simulink library "multicopterNDI_lib"  (R2018b)
settings: Solver=VariableStepAuto  StartTime=0.0  StopTime=10.0  RelTol=1e-3
undefined symbols (not defined in the file or in its folder): cntrl, DiscIntNeverNeededParam
libraries: ndi_lib x5, axes_transformation_lib x1
settings Model: Creator=Ybeyer  LastModifiedBy=yannic
settings SFSimCC: SimUseLocalCustomCode=off
settings RTWCC: RTWUseLocalCustomCode=off
settings CodeAppCC: StateflowObjectComments=on

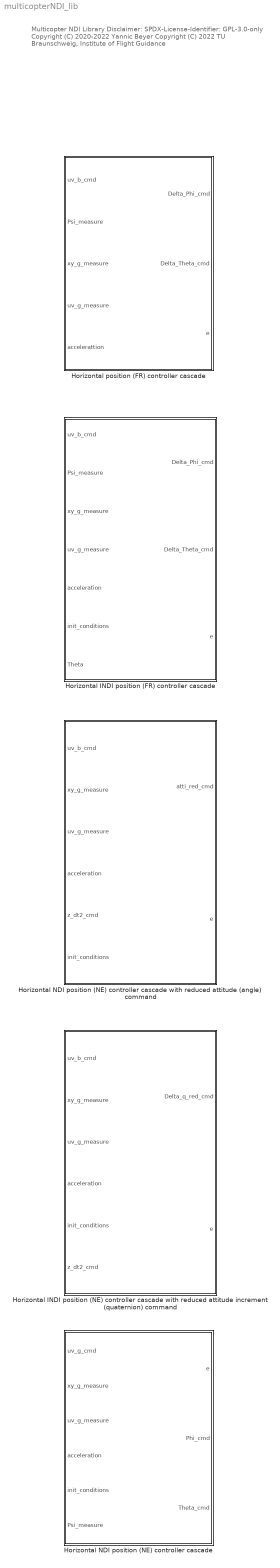
== system multicopterNDI_lib ==
  note: Multicopter NDI Library
      |
      | Disclaimer:
      | SPDX-License-Identifier: GPL-3.0-only
      |
      | Copyright (C) 2020-2022 Yannic Beyer
      | Copyright (C) 2022 TU Braunschweig, Institute of Flight Guidance
  Horizontal INDI position (FR) controller cascade : Subsystem  mask{time_constant_V=cntrl.rm.u.T, V_dt_max=inf, K_xyuv=cntrl.Kpos, K_int_xy=zeros(2,2), Phi_cmd_max=pi/4, Theta_cmd_max=pi/4}
      mask prompts: time_constant_V "commanded velocity time constant, in s"; V_dt_max "maximum commanded acceleration"; K_xyuv "controller matrix [e_x,e_y,e_u,e_v] -> [x_ddt,y_ddt]_cmd"; K_int_xy "I controller matrix [int_e_x,int_e_y] -> [x_ddt,y_ddt]_cmd"; Phi_cmd_max "Maximum commanded roll angle"; Theta_cmd_max "Maximum commanded picth angle"
      mask DialogControl DescGroupVar Prompt: Horizontal position controller cascade
      mask DialogControl DescTextVar Prompt: The commanded velocity is filtered and the control error is converted into desired accerlations in x_b and y_b direction. The commanded accelerations are converted into commanded roll and pitch angles.
  Horizontal INDI position (NE) controller cascade with reduced attitude increment (quaternion) command : Subsystem  mask{time_constant_V=cntrl.rm.u.T, V_dt_max=cntrl.rm.uv_dt_max, K_xyuv=cntrl.Kpos, tilt_angle_max=cntrl.rm.Phi_max, e_xy_max=cntrl.e_xy_max}
      mask prompts: time_constant_V "commanded velocity time constant, in s"; V_dt_max "maximum commanded acceleration"; K_xyuv "controller matrix [e_x,e_y,e_u,e_v] -> [x_ddt,y_ddt]_cmd"; tilt_angle_max "Maximum commanded tilt angle"; e_xy_max "Maximum position error (to limit maximum velocity due to controller)"
      mask DialogControl DescGroupVar Prompt: Horizontal position controller cascade
      mask DialogControl DescTextVar Prompt: The commanded velocity is filtered and the control error is converted into desired accerlations in x_b and y_b direction. The commanded accelerations are converted into commanded roll and pitch angles.
  Horizontal NDI position (NE) controller cascade : Subsystem  mask{time_constant_V=cntrl.rm.u.T, V_dt_max=inf, K_xyuv=cntrl.Kpos, K_int_xy=zeros(2,2), Phi_cmd_max=pi/4, Theta_cmd_max=pi/4}
      mask prompts: time_constant_V "commanded velocity time constant, in s"; V_dt_max "maximum commanded acceleration"; K_xyuv "controller matrix [e_x,e_y,e_u,e_v] -> [x_ddt,y_ddt]_cmd"; K_int_xy "I controller matrix [int_e_x,int_e_y] -> [x_ddt,y_ddt]_cmd"; Phi_cmd_max "Maximum commanded roll angle"; Theta_cmd_max "Maximum commanded picth angle"
      mask DialogControl DescGroupVar Prompt: Horizontal position controller cascade (commanding velocities/positions in north/east (NE) direction)
      mask DialogControl DescTextVar Prompt: The commanded velocity is filtered and the control error is converted into desired accerlations in x_b and y_b direction. The commanded accelerations are converted into commanded roll and pitch angles.
  Horizontal NDI position (NE) controller cascade with reduced attitude (angle) command : Subsystem  mask{time_constant_V=cntrl.rm.u.T, V_dt_max=cntrl.rm.uv_dt_max, K_xyuv=cntrl.Kpos, K_int_xy=cntrl.Kpos_I, e_xy_max=cntrl.e_xy_max}
      mask prompts: time_constant_V "commanded velocity time constant, in s"; V_dt_max "maximum commanded acceleration"; K_xyuv "controller matrix [e_x,e_y,e_u,e_v] -> [x_ddt,y_ddt]_cmd"; K_int_xy "I controller matrix [int_e_x,int_e_y] -> [x_ddt,y_ddt]_cmd"; e_xy_max "Maximum controller position error (to limit maximum velocity due to controller)"
      mask DialogControl DescGroupVar Prompt: Horizontal position controller cascade
      mask DialogControl DescTextVar Prompt: The commanded velocity is filtered and the control error is converted into desired accerlations in x_g and y_g direction. The commanded accelerations are converted into commanded to reduced attitude angles.
  Horizontal position (FR) controller cascade : Subsystem  mask{time_constant_V=1, V_dt_max=inf, K_xyuv=zeros(2,4), K_int_xy=zeros(2,2), Phi_cmd_max=pi/4, Theta_cmd_max=pi/4}
      mask prompts: time_constant_V "commanded velocity time constant, in s"; V_dt_max "maximum commanded acceleration"; K_xyuv "controller matrix [e_x,e_y,e_u,e_v] -> [x_ddt,y_ddt]_cmd"; K_int_xy "I controller matrix [int_e_x,int_e_y] -> [x_ddt,y_ddt]_cmd"; Phi_cmd_max "Maximum commanded roll angle"; Theta_cmd_max "Maximum commanded picth angle"
      mask DialogControl DescGroupVar Prompt: Horizontal position controller cascade
      mask DialogControl DescTextVar Prompt: The commanded velocity is filtered and the control error is converted into desired accerlations in x_b and y_b direction. The commanded accelerations are converted into commanded roll and pitch angles.

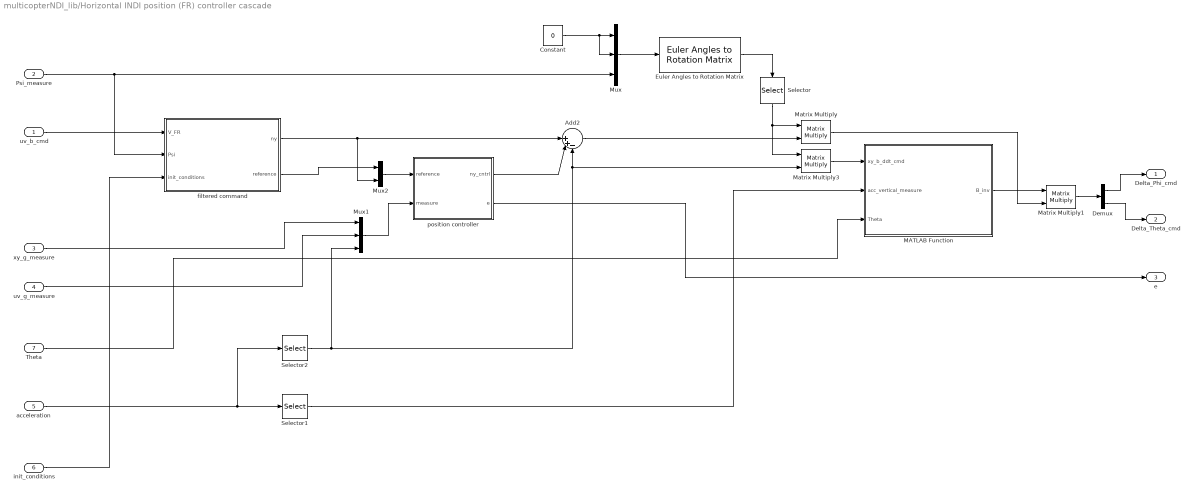
== system multicopterNDI_lib/Horizontal INDI position (FR) controller cascade ==
  uv_b_cmd : Inport
  Psi_measure : Inport  Port=2
  xy_g_measure : Inport  Port=3
  uv_g_measure : Inport  Port=4
  acceleration : Inport  Port=5
  init_conditions : Inport  Port=6
  Theta : Inport  Port=7
  Add2 : Sum  Inputs=||++-
  Constant : Constant  Value=0  OutDataTypeStr=Inherit: Inherit via back propagation
  Demux : Demux  Outputs=2
  Euler Angles to Rotation Matrix : axes_transformation_lib/Euler Angles to Rotation Matrix  SystemSampleTime=-1
      settings: SourceProductName=LADAC
  MATLAB Function : MATLAB Function  TreatAsAtomicUnit=on
  Matrix Multiply : Product  Multiplication=Matrix(*)
  Matrix Multiply1 : Product  Multiplication=Matrix(*)
  Matrix Multiply3 : Product  Multiplication=Matrix(*)
  Mux : Mux  Inputs=3
  Mux1 : Mux  Inputs=3
  Mux2 : Mux  Inputs=2
  Selector : Selector  NumberOfDimensions=2  InputPortWidth=[3,3]  IndexOptions=Index vector (dialog),Index vector (dialog)  Indices=[1:2],[1:2]  OutputSizes=1,1
  Selector1 : Selector  InputPortWidth=3  IndexOptions=Index vector (dialog)  Indices=3  OutputSizes=1
  Selector2 : Selector  InputPortWidth=3  IndexOptions=Index vector (dialog)  Indices=[1,2]  OutputSizes=1
  filtered command : Subsystem
  position controller : Subsystem
  Delta_Phi_cmd : Outport
  Delta_Theta_cmd : Outport  Port=2
  e : Outport  Port=3
  wires:
  init_conditions/1 -> filtered command/3(init_conditions)
  Mux2/1 -> position controller/1(reference)
  position controller/2(e) -> e/1
  Matrix Multiply1/1 -> Demux/1
  Demux/2 -> Delta_Theta_cmd/1
  Demux/1 -> Delta_Phi_cmd/1
  MATLAB Function/1(B_inv) -> Matrix Multiply1/1
  Selector2/1 -> Mux1/3, Add2/3, Matrix Multiply3/2
  Selector1/1 -> MATLAB Function/2(acc_vertical_measure)
  Euler Angles to Rotation Matrix/1 -> Selector/1
  Matrix Multiply/1 -> Matrix Multiply1/2
  Constant/1 -> Mux/1, Mux/2
  Mux/1 -> Euler Angles to Rotation Matrix/1
  Psi_measure/1 -> filtered command/2(Psi), Mux/3
  filtered command/2(reference) -> Mux2/1
  uv_b_cmd/1 -> filtered command/1(V_FR)
  acceleration/1 -> Selector2/1, Selector1/1
  position controller/1(ny_cntrl) -> Add2/2
  filtered command/1(ny) -> Mux2/2, Add2/1
  Add2/1 -> Matrix Multiply/2
  Mux1/1 -> position controller/2(measure)
  xy_g_measure/1 -> Mux1/1
  uv_g_measure/1 -> Mux1/2
  Matrix Multiply3/1 -> MATLAB Function/1(xy_b_ddt_cmd)
  Selector/1 -> Matrix Multiply3/1, Matrix Multiply/1
  Theta/1 -> MATLAB Function/3(Theta)

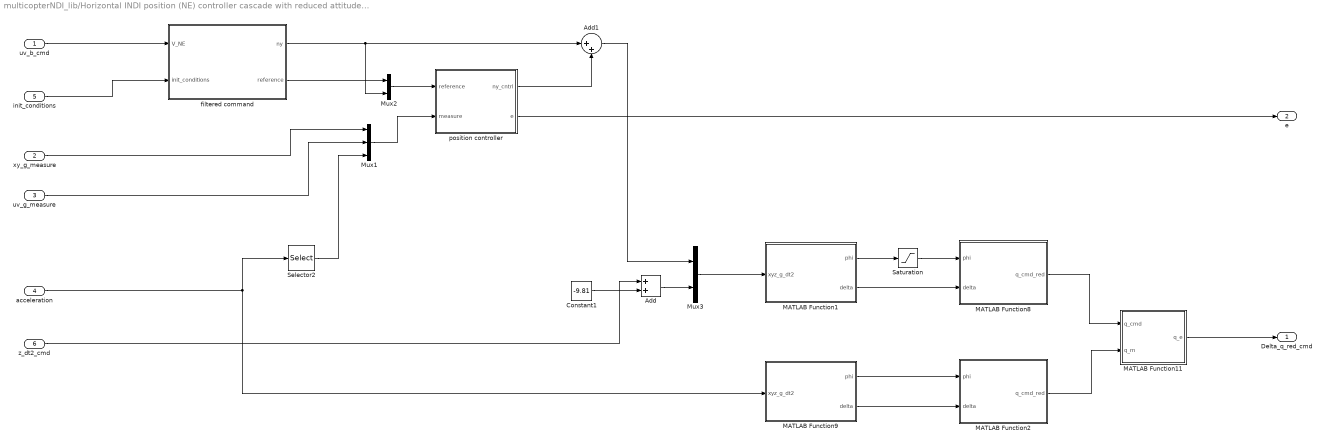
== system multicopterNDI_lib/Horizontal INDI position (NE) controller cascade with reduced attitude increment (quaternion) command ==
  uv_b_cmd : Inport
  xy_g_measure : Inport  Port=2
  uv_g_measure : Inport  Port=3
  acceleration : Inport  Port=4
  init_conditions : Inport  Port=5
  z_dt2_cmd : Inport  Port=6
  Add : Sum
  Add1 : Sum  Inputs=|++
  Constant1 : Constant  Value=-9.81  OutDataTypeStr=single
  MATLAB Function1 : MATLAB Function  TreatAsAtomicUnit=on
  MATLAB Function11 : MATLAB Function  TreatAsAtomicUnit=on
  MATLAB Function2 : MATLAB Function  TreatAsAtomicUnit=on
  MATLAB Function8 : MATLAB Function  TreatAsAtomicUnit=on
  MATLAB Function9 : MATLAB Function  TreatAsAtomicUnit=on
  Mux1 : Mux  Inputs=3
  Mux2 : Mux  Inputs=2
  Mux3 : Mux  Inputs=2
  Saturation : Saturate  UpperLimit=tilt_angle_max  LowerLimit=0
  Selector2 : Selector  InputPortWidth=3  IndexOptions=Index vector (dialog)  Indices=[1,2]  OutputSizes=1
  filtered command : Subsystem
  position controller : Subsystem
  Delta_q_red_cmd : Outport
  e : Outport  Port=2
  wires:
  uv_g_measure/1 -> Mux1/2
  xy_g_measure/1 -> Mux1/1
  Mux1/1 -> position controller/2(measure)
  filtered command/1(ny) -> Add1/1, Mux2/2
  uv_b_cmd/1 -> filtered command/1(V_NE)
  filtered command/2(reference) -> Mux2/1
  Selector2/1 -> Mux1/3
  position controller/2(e) -> e/1
  Mux2/1 -> position controller/1(reference)
  init_conditions/1 -> filtered command/2(init_conditions)
  z_dt2_cmd/1 -> Add/1
  MATLAB Function1/1(phi) -> Saturation/1
  MATLAB Function1/2(delta) -> MATLAB Function8/2(delta)
  position controller/1(ny_cntrl) -> Add1/2
  acceleration/1 -> MATLAB Function9/1(xyz_g_dt2), Selector2/1
  MATLAB Function9/1(phi) -> MATLAB Function2/1(phi)
  MATLAB Function9/2(delta) -> MATLAB Function2/2(delta)
  MATLAB Function8/1(q_cmd_red) -> MATLAB Function11/1(q_cmd)
  MATLAB Function2/1(q_cmd_red) -> MATLAB Function11/2(q_m)
  MATLAB Function11/1(q_e) -> Delta_q_red_cmd/1
  Add/1 -> Mux3/2
  Constant1/1 -> Add/2
  Mux3/1 -> MATLAB Function1/1(xyz_g_dt2)
  Add1/1 -> Mux3/1
  Saturation/1 -> MATLAB Function8/1(phi)

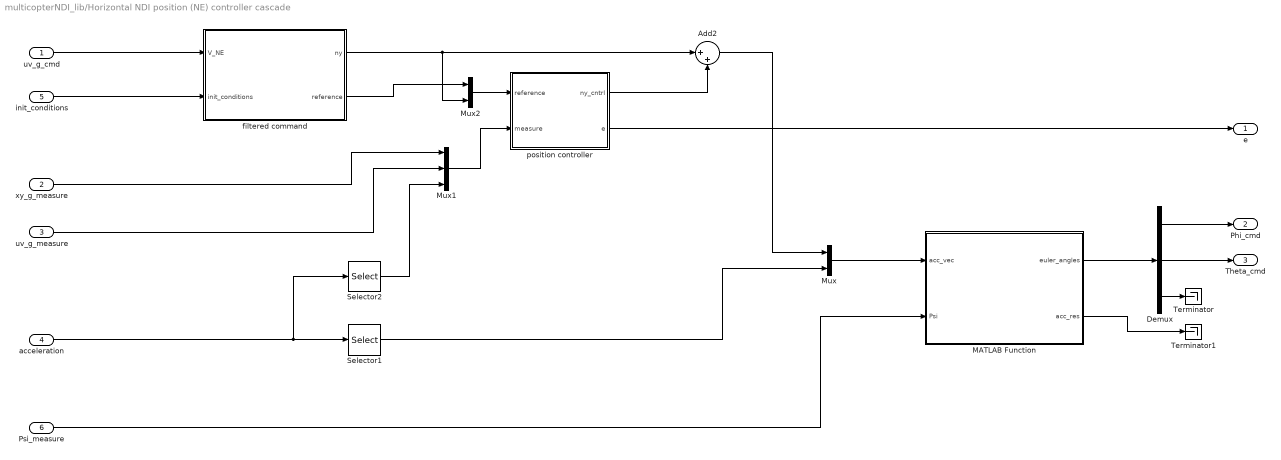
== system multicopterNDI_lib/Horizontal NDI position (NE) controller cascade ==
  uv_g_cmd : Inport
  xy_g_measure : Inport  Port=2
  uv_g_measure : Inport  Port=3
  acceleration : Inport  Port=4
  init_conditions : Inport  Port=5
  Psi_measure : Inport  Port=6
  Add2 : Sum  Inputs=|++
  Demux : Demux  Outputs=3
  MATLAB Function : MATLAB Function  TreatAsAtomicUnit=on
  Mux : Mux  Inputs=2
  Mux1 : Mux  Inputs=3
  Mux2 : Mux  Inputs=2
  Selector1 : Selector  InputPortWidth=3  IndexOptions=Index vector (dialog)  Indices=3  OutputSizes=1
  Selector2 : Selector  InputPortWidth=3  IndexOptions=Index vector (dialog)  Indices=[1,2]  OutputSizes=1
  Terminator : Terminator
  Terminator1 : Terminator
  filtered command : Subsystem
  position controller : Subsystem
  e : Outport
  Phi_cmd : Outport  Port=2
  Theta_cmd : Outport  Port=3
  wires:
  init_conditions/1 -> filtered command/2(init_conditions)
  Mux2/1 -> position controller/1(reference)
  position controller/2(e) -> e/1
  Selector2/1 -> Mux1/3
  Selector1/1 -> Mux/2
  filtered command/2(reference) -> Mux2/1
  uv_g_cmd/1 -> filtered command/1(V_NE)
  acceleration/1 -> Selector2/1, Selector1/1
  position controller/1(ny_cntrl) -> Add2/2
  filtered command/1(ny) -> Mux2/2, Add2/1
  Add2/1 -> Mux/1
  Mux1/1 -> position controller/2(measure)
  xy_g_measure/1 -> Mux1/1
  uv_g_measure/1 -> Mux1/2
  Demux/1 -> Phi_cmd/1
  Demux/2 -> Theta_cmd/1
  Psi_measure/1 -> MATLAB Function/2(Psi)
  Mux/1 -> MATLAB Function/1(acc_vec)
  MATLAB Function/1(euler_angles) -> Demux/1
  Demux/3 -> Terminator/1
  MATLAB Function/2(acc_res) -> Terminator1/1

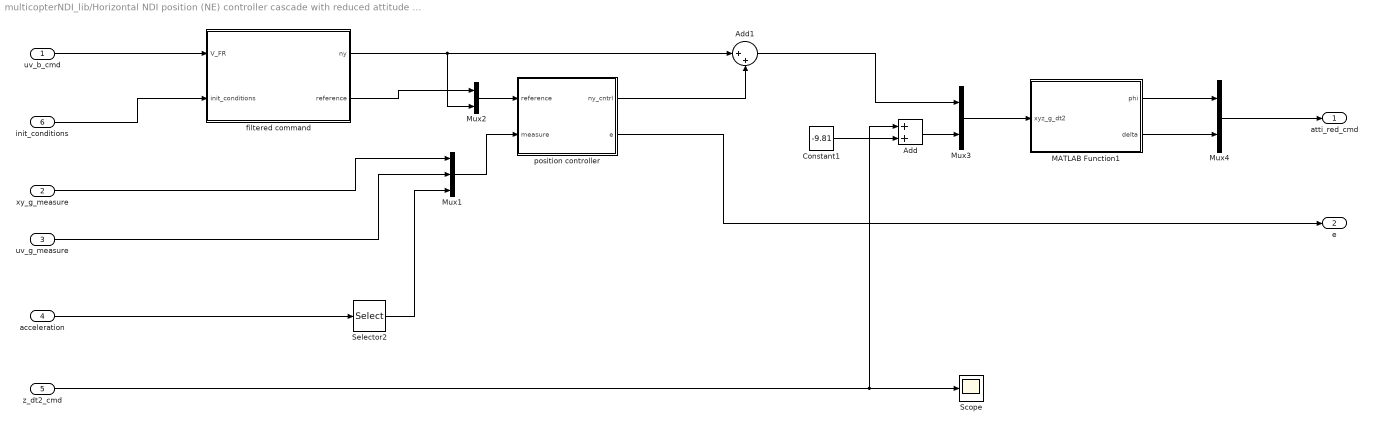
== system multicopterNDI_lib/Horizontal NDI position (NE) controller cascade with reduced attitude (angle) command ==
  uv_b_cmd : Inport
  xy_g_measure : Inport  Port=2
  uv_g_measure : Inport  Port=3
  acceleration : Inport  Port=4
  z_dt2_cmd : Inport  Port=5
  init_conditions : Inport  Port=6
  Add : Sum
  Add1 : Sum  Inputs=|++
  Constant1 : Constant  Value=-9.81  OutDataTypeStr=single
  MATLAB Function1 : MATLAB Function  TreatAsAtomicUnit=on
  Mux1 : Mux  Inputs=3
  Mux2 : Mux  Inputs=2
  Mux3 : Mux  Inputs=2
  Mux4 : Mux  Inputs=2
  Scope : Scope
  Selector2 : Selector  InputPortWidth=3  IndexOptions=Index vector (dialog)  Indices=[1,2]  OutputSizes=1
  filtered command : Subsystem
  position controller : Subsystem
  atti_red_cmd : Outport
  e : Outport  Port=2
  wires:
  uv_g_measure/1 -> Mux1/2
  xy_g_measure/1 -> Mux1/1
  Mux1/1 -> position controller/2(measure)
  filtered command/1(ny) -> Add1/1, Mux2/2
  uv_b_cmd/1 -> filtered command/1(V_FR)
  filtered command/2(reference) -> Mux2/1
  Selector2/1 -> Mux1/3
  position controller/2(e) -> e/1
  Mux2/1 -> position controller/1(reference)
  init_conditions/1 -> filtered command/2(init_conditions)
  z_dt2_cmd/1 -> Scope/1, Add/1
  MATLAB Function1/1(phi) -> Mux4/1
  MATLAB Function1/2(delta) -> Mux4/2
  position controller/1(ny_cntrl) -> Add1/2
  acceleration/1 -> Selector2/1
  Add/1 -> Mux3/2
  Constant1/1 -> Add/2
  Mux3/1 -> MATLAB Function1/1(xyz_g_dt2)
  Add1/1 -> Mux3/1
  Mux4/1 -> atti_red_cmd/1

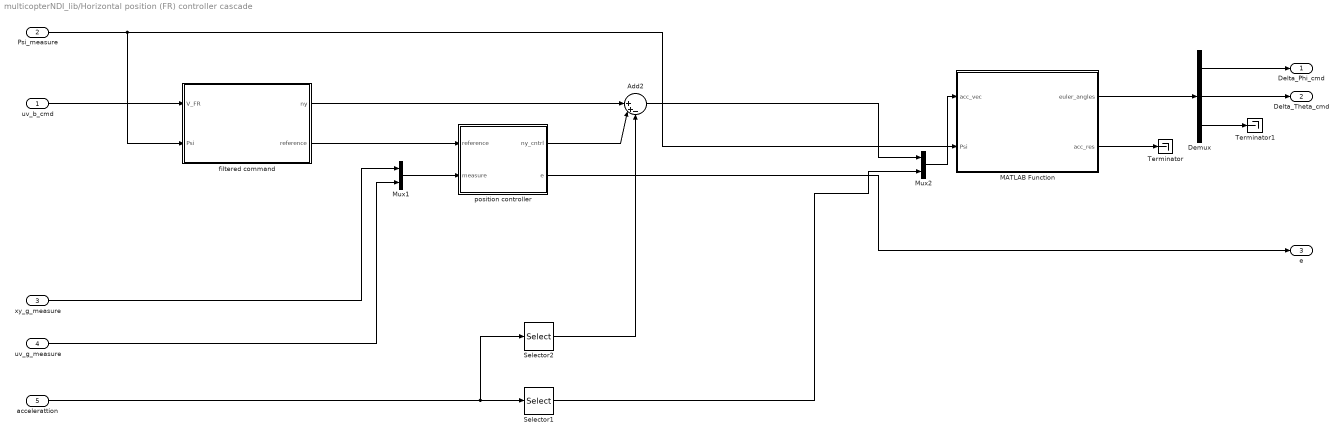
== system multicopterNDI_lib/Horizontal position (FR) controller cascade ==
  uv_b_cmd : Inport
  Psi_measure : Inport  Port=2
  xy_g_measure : Inport  Port=3
  uv_g_measure : Inport  Port=4
  accelerattion : Inport  Port=5
  Add2 : Sum  Inputs=||++-
  Demux : Demux  Outputs=3
  MATLAB Function : MATLAB Function  TreatAsAtomicUnit=on
  Mux1 : Mux  Inputs=2
  Mux2 : Mux  Inputs=2
  Selector1 : Selector  InputPortWidth=3  IndexOptions=Index vector (dialog)  Indices=3  OutputSizes=1
  Selector2 : Selector  InputPortWidth=3  IndexOptions=Index vector (dialog)  Indices=[1,2]  OutputSizes=1
  Terminator : Terminator
  Terminator1 : Terminator
  filtered command : Subsystem
  position controller : Subsystem
  Delta_Phi_cmd : Outport
  Delta_Theta_cmd : Outport  Port=2
  e : Outport  Port=3
  wires:
  position controller/2(e) -> e/1
  MATLAB Function/1(euler_angles) -> Demux/1
  Demux/2 -> Delta_Theta_cmd/1
  Demux/1 -> Delta_Phi_cmd/1
  Selector2/1 -> Add2/3
  Selector1/1 -> Mux2/2
  Psi_measure/1 -> filtered command/2(Psi), MATLAB Function/2(Psi)
  filtered command/2(reference) -> position controller/1(reference)
  uv_b_cmd/1 -> filtered command/1(V_FR)
  accelerattion/1 -> Selector1/1, Selector2/1
  position controller/1(ny_cntrl) -> Add2/2
  filtered command/1(ny) -> Add2/1
  Add2/1 -> Mux2/1
  Mux1/1 -> position controller/2(measure)
  xy_g_measure/1 -> Mux1/1
  uv_g_measure/1 -> Mux1/2
  MATLAB Function/2(acc_res) -> Terminator/1
  Mux2/1 -> MATLAB Function/1(acc_vec)
  Demux/3 -> Terminator1/1

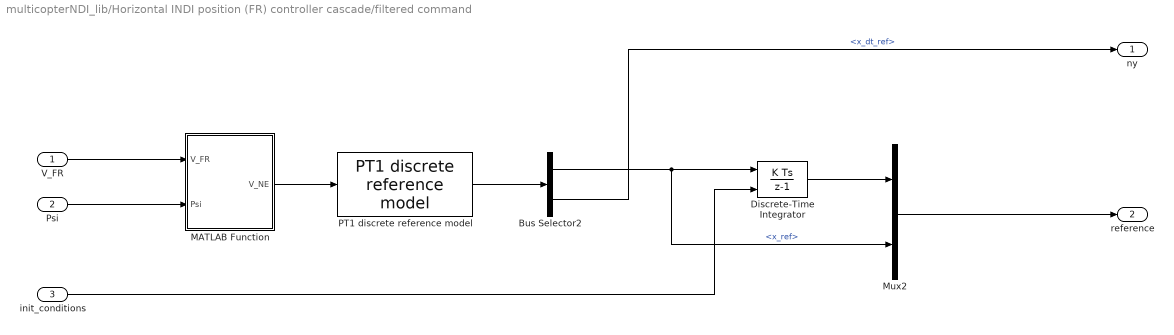
== system multicopterNDI_lib/Horizontal INDI position (FR) controller cascade/filtered command ==
  V_FR : Inport
  Psi : Inport  Port=2
  init_conditions : Inport  Port=3
  Bus Selector2 : BusSelector  OutputSignals=x_ref,x_dt_ref
  Discrete-Time Integrator : DiscreteIntegrator  InitialConditionSource=external  SampleTime=-1  ICPrevOutput=DiscIntNeverNeededParam  ICPrevScaledInput=DiscIntNeverNeededParam
  MATLAB Function : MATLAB Function  TreatAsAtomicUnit=on
  Mux2 : Mux  Inputs=2
  PT1 discrete reference model : ndi_lib/PT1 discrete reference model  T=time_constant_V  x_max=inf  x_min=-inf  x_dt_max=V_dt_max  x_dt_min=-V_dt_max  x_init=0
      settings: SourceProductName=LADAC
  ny : Outport
  reference : Outport  Port=2
  wires:
  init_conditions/1 -> Discrete-Time Integrator/2
  Psi/1 -> MATLAB Function/2(Psi)
  Bus Selector2/2 -> ny/1  "<x_dt_ref>"
  Bus Selector2/1 -> Mux2/2, Discrete-Time Integrator/1  "<x_ref>"
  Discrete-Time Integrator/1 -> Mux2/1
  PT1 discrete reference model/1 -> Bus Selector2/1
  Mux2/1 -> reference/1
  V_FR/1 -> MATLAB Function/1(V_FR)
  MATLAB Function/1(V_NE) -> PT1 discrete reference model/1

== system multicopterNDI_lib/Horizontal INDI position (FR) controller cascade/position controller ==
  reference : Inport
  measure : Inport  Port=2
  Add : Sum  Inputs=+-
  Gain : Gain  Gain=K_xyuv  Multiplication=Matrix(K*u)
  ny_cntrl : Outport
  e : Outport  Port=2
  wires:
  Gain/1 -> ny_cntrl/1
  Add/1 -> Gain/1, e/1
  measure/1 -> Add/2
  reference/1 -> Add/1

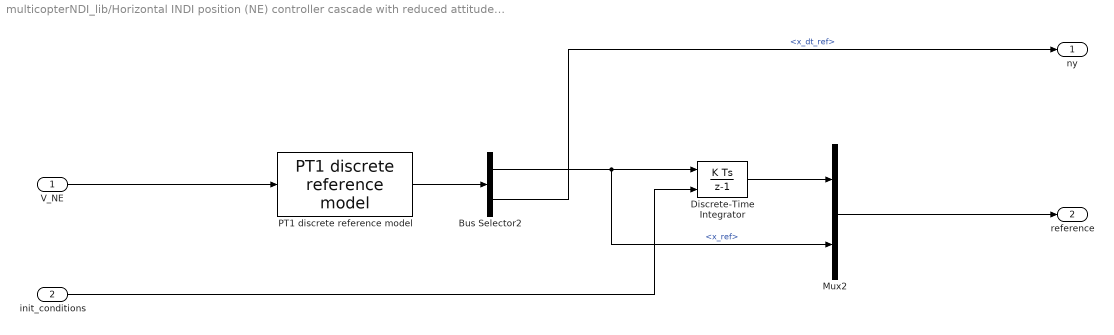
== system multicopterNDI_lib/Horizontal INDI position (NE) controller cascade with reduced attitude increment (quaternion) command/filtered command ==
  V_NE : Inport
  init_conditions : Inport  Port=2
  Bus Selector2 : BusSelector  OutputSignals=x_ref,x_dt_ref
  Discrete-Time Integrator : DiscreteIntegrator  InitialConditionSource=external  SampleTime=-1  ICPrevOutput=DiscIntNeverNeededParam  ICPrevScaledInput=DiscIntNeverNeededParam
  Mux2 : Mux  Inputs=2
  PT1 discrete reference model : ndi_lib/PT1 discrete reference model  T=time_constant_V  x_max=inf  x_min=-inf  x_dt_max=V_dt_max  x_dt_min=-V_dt_max  x_init=0
      settings: SourceProductName=LADAC
  ny : Outport
  reference : Outport  Port=2
  wires:
  V_NE/1 -> PT1 discrete reference model/1
  Mux2/1 -> reference/1
  PT1 discrete reference model/1 -> Bus Selector2/1
  Discrete-Time Integrator/1 -> Mux2/1
  Bus Selector2/1 -> Discrete-Time Integrator/1, Mux2/2  "<x_ref>"
  Bus Selector2/2 -> ny/1  "<x_dt_ref>"
  init_conditions/1 -> Discrete-Time Integrator/2

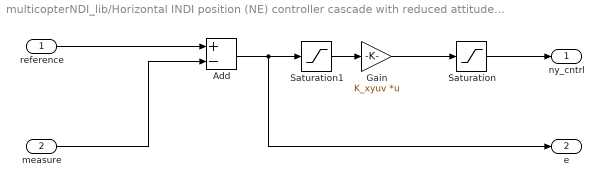
== system multicopterNDI_lib/Horizontal INDI position (NE) controller cascade with reduced attitude increment (quaternion) command/position controller ==
  reference : Inport
  measure : Inport  Port=2
  Add : Sum  Inputs=+-
  Gain : Gain  Gain=K_xyuv  Multiplication=Matrix(K*u)
  Saturation : Saturate  UpperLimit=cntrl.rm.uv_dt_max  LowerLimit=-cntrl.rm.uv_dt_max
  Saturation1 : Saturate  UpperLimit=[e_xy_max;1000;1000;1000;1000]  LowerLimit=-[e_xy_max;1000;1000;1000;1000]
  ny_cntrl : Outport
  e : Outport  Port=2
  wires:
  reference/1 -> Add/1
  measure/1 -> Add/2
  Gain/1 -> Saturation/1
  Add/1 -> Saturation1/1, e/1
  Saturation/1 -> ny_cntrl/1
  Saturation1/1 -> Gain/1

== system multicopterNDI_lib/Horizontal NDI position (NE) controller cascade/filtered command ==
  V_NE : Inport
  init_conditions : Inport  Port=2
  Bus Selector2 : BusSelector  OutputSignals=x_ref,x_dt_ref
  Discrete-Time Integrator : DiscreteIntegrator  InitialConditionSource=external  SampleTime=-1  ICPrevOutput=DiscIntNeverNeededParam  ICPrevScaledInput=DiscIntNeverNeededParam
  Mux2 : Mux  Inputs=2
  PT1 discrete reference model : ndi_lib/PT1 discrete reference model  T=time_constant_V  x_max=inf  x_min=-inf  x_dt_max=V_dt_max  x_dt_min=-V_dt_max  x_init=0
      settings: SourceProductName=LADAC
  ny : Outport
  reference : Outport  Port=2
  wires:
  init_conditions/1 -> Discrete-Time Integrator/2
  Bus Selector2/2 -> ny/1  "<x_dt_ref>"
  Bus Selector2/1 -> Mux2/2, Discrete-Time Integrator/1  "<x_ref>"
  Discrete-Time Integrator/1 -> Mux2/1
  PT1 discrete reference model/1 -> Bus Selector2/1
  Mux2/1 -> reference/1
  V_NE/1 -> PT1 discrete reference model/1

== system multicopterNDI_lib/Horizontal NDI position (NE) controller cascade/position controller ==
  reference : Inport
  measure : Inport  Port=2
  Add : Sum  Inputs=+-
  Gain : Gain  Gain=K_xyuv  Multiplication=Matrix(K*u)
  ny_cntrl : Outport
  e : Outport  Port=2
  wires:
  Gain/1 -> ny_cntrl/1
  Add/1 -> Gain/1, e/1
  measure/1 -> Add/2
  reference/1 -> Add/1

== system multicopterNDI_lib/Horizontal NDI position (NE) controller cascade with reduced attitude (angle) command/filtered command ==
  V_FR : Inport
  init_conditions : Inport  Port=2
  Bus Selector2 : BusSelector  OutputSignals=x_ref,x_dt_ref
  Discrete-Time Integrator : DiscreteIntegrator  InitialConditionSource=external  SampleTime=-1  ICPrevOutput=DiscIntNeverNeededParam  ICPrevScaledInput=DiscIntNeverNeededParam
  Mux2 : Mux  Inputs=2
  PT1 discrete reference model : ndi_lib/PT1 discrete reference model  T=time_constant_V  x_max=inf  x_min=-inf  x_dt_max=V_dt_max  x_dt_min=-V_dt_max  x_init=0
      settings: SourceProductName=LADAC
  ny : Outport
  reference : Outport  Port=2
  wires:
  V_FR/1 -> PT1 discrete reference model/1
  Mux2/1 -> reference/1
  PT1 discrete reference model/1 -> Bus Selector2/1
  Discrete-Time Integrator/1 -> Mux2/1
  Bus Selector2/1 -> Discrete-Time Integrator/1, Mux2/2  "<x_ref>"
  Bus Selector2/2 -> ny/1  "<x_dt_ref>"
  init_conditions/1 -> Discrete-Time Integrator/2

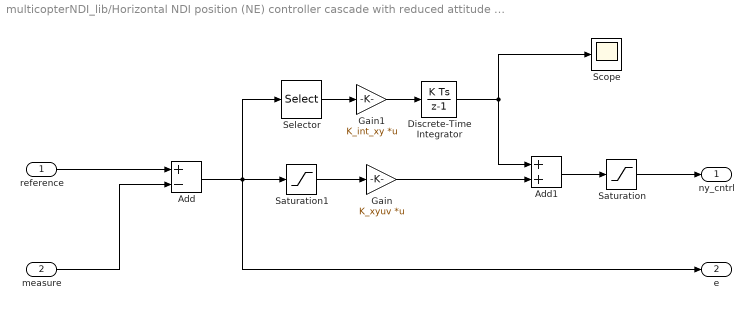
== system multicopterNDI_lib/Horizontal NDI position (NE) controller cascade with reduced attitude (angle) command/position controller ==
  reference : Inport
  measure : Inport  Port=2
  Add : Sum  Inputs=+-
  Add1 : Sum
  Discrete-Time Integrator : DiscreteIntegrator  SampleTime=-1  LimitOutput=on  UpperSaturationLimit=e_xy_max  LowerSaturationLimit=-e_xy_max  ICPrevOutput=DiscIntNeverNeededParam  ICPrevScaledInput=DiscIntNeverNeededParam
  Gain : Gain  Gain=K_xyuv  Multiplication=Matrix(K*u)
  Gain1 : Gain  Gain=K_int_xy  Multiplication=Matrix(K*u)
  Saturation : Saturate  UpperLimit=cntrl.rm.uv_dt_max  LowerLimit=-cntrl.rm.uv_dt_max
  Saturation1 : Saturate  UpperLimit=[e_xy_max;inf;inf;inf;inf]  LowerLimit=-[e_xy_max;inf;inf;inf;inf]
  Scope : Scope
  Selector : Selector  InputPortWidth=6  IndexOptions=Index vector (dialog)  Indices=[1:2]  OutputSizes=1
  ny_cntrl : Outport
  e : Outport  Port=2
  wires:
  reference/1 -> Add/1
  measure/1 -> Add/2
  Gain/1 -> Add1/2
  Add/1 -> Selector/1, Saturation1/1, e/1
  Saturation/1 -> ny_cntrl/1
  Saturation1/1 -> Gain/1
  Selector/1 -> Gain1/1
  Add1/1 -> Saturation/1
  Discrete-Time Integrator/1 -> Scope/1, Add1/1
  Gain1/1 -> Discrete-Time Integrator/1

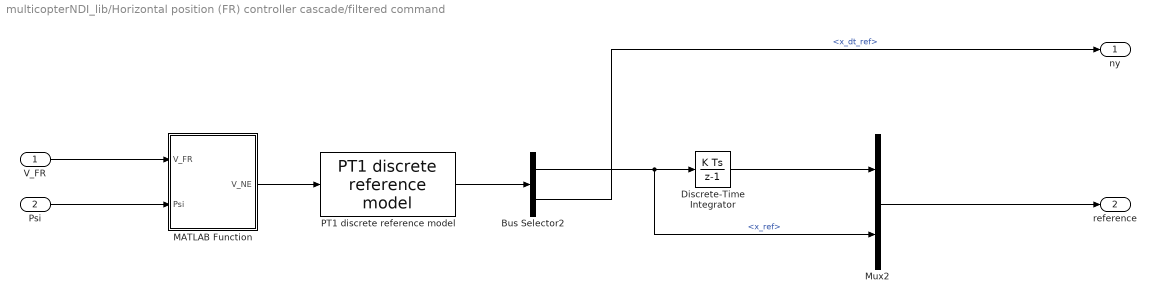
== system multicopterNDI_lib/Horizontal position (FR) controller cascade/filtered command ==
  V_FR : Inport
  Psi : Inport  Port=2
  Bus Selector2 : BusSelector  OutputSignals=x_ref,x_dt_ref
  Discrete-Time Integrator : DiscreteIntegrator  SampleTime=-1  ICPrevOutput=DiscIntNeverNeededParam  ICPrevScaledInput=DiscIntNeverNeededParam
  MATLAB Function : MATLAB Function  TreatAsAtomicUnit=on
  Mux2 : Mux  Inputs=2
  PT1 discrete reference model : ndi_lib/PT1 discrete reference model  T=time_constant_V  x_max=inf  x_min=-inf  x_dt_max=V_dt_max  x_dt_min=-V_dt_max  x_init=0
      settings: SourceProductName=LADAC
  ny : Outport
  reference : Outport  Port=2
  wires:
  Psi/1 -> MATLAB Function/2(Psi)
  MATLAB Function/1(V_NE) -> PT1 discrete reference model/1
  Bus Selector2/2 -> ny/1  "<x_dt_ref>"
  Bus Selector2/1 -> Mux2/2, Discrete-Time Integrator/1  "<x_ref>"
  Discrete-Time Integrator/1 -> Mux2/1
  PT1 discrete reference model/1 -> Bus Selector2/1
  V_FR/1 -> MATLAB Function/1(V_FR)
  Mux2/1 -> reference/1

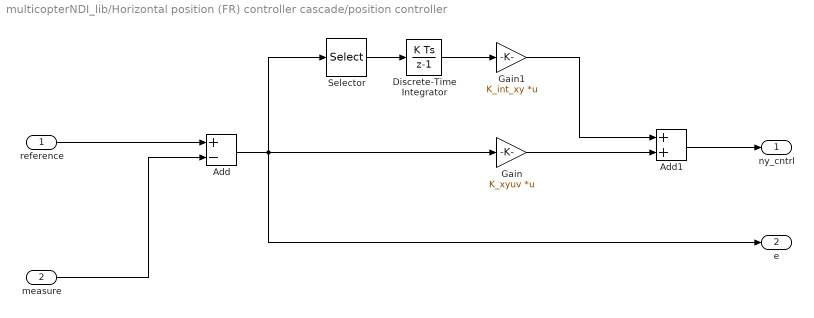
== system multicopterNDI_lib/Horizontal position (FR) controller cascade/position controller ==
  reference : Inport
  measure : Inport  Port=2
  Add : Sum  Inputs=+-
  Add1 : Sum
  Discrete-Time Integrator : DiscreteIntegrator  SampleTime=-1  ICPrevOutput=DiscIntNeverNeededParam  ICPrevScaledInput=DiscIntNeverNeededParam
  Gain : Gain  Gain=K_xyuv  Multiplication=Matrix(K*u)
  Gain1 : Gain  Gain=K_int_xy  Multiplication=Matrix(K*u)
  Selector : Selector  InputPortWidth=4  IndexOptions=Index vector (dialog)  Indices=[1,2]  OutputSizes=1
  ny_cntrl : Outport
  e : Outport  Port=2
  wires:
  Gain1/1 -> Add1/1
  Discrete-Time Integrator/1 -> Gain1/1
  Add1/1 -> ny_cntrl/1
  Selector/1 -> Discrete-Time Integrator/1
  Add/1 -> Gain/1, Selector/1, e/1
  Gain/1 -> Add1/2
  measure/1 -> Add/2
  reference/1 -> Add/1

== matlab function multicopterNDI_lib/Horizontal INDI position (NE) controller cascade with reduced attitude increment (quaternion) command/MATLAB Function1 ==
  data: phi output; delta output; xyz_g_dt2 input
function [phi,delta] = fcn(xyz_g_dt2)
% function [x,y] = fcn(xyz_g_dt2)

if abs(xyz_g_dt2(3)) < 1
    if xyz_g_dt2(3) > 0
        xyz_g_dt2(3) = 1;
    else
        xyz_g_dt2(3) = -1;
    end
end

% x = atan2(xyz_g_dt2(1),-xyz_g_dt2(3));
% y = atan2(xyz_g_dt2(2),-xyz_g_dt2(3));


delta = atan2(xyz_g_dt2(2),xyz_g_dt2(1));
xy_g_dt2 = sqrt( xyz_g_dt2(1)^2 + xyz_g_dt2(2)^2 );
phi = atan2( xy_g_dt2 , -xyz_g_dt2(3) );

end

== matlab function multicopterNDI_lib/Horizontal position (FR) controller cascade/MATLAB Function ==
  data: acc_vec input; euler_angles output; Psi input; acc_res output
function [euler_angles, acc_res] = fcn(acc_vec, Psi) %#codegen
[euler_angles, acc_res] = ...
    getEulerAnglesFromAccelerationVectorAndHeading(acc_vec, Psi);
end

== matlab function multicopterNDI_lib/Horizontal position (FR) controller cascade/filtered command/MATLAB Function ==
  data: V_FR input; V_NE output; Psi input
function V_NE = fcn(V_FR,Psi)

V_NE = [ cos(Psi), -sin(Psi); sin(Psi), cos(Psi) ] * V_FR;

end

== matlab function multicopterNDI_lib/Horizontal NDI position (NE) controller cascade/MATLAB Function ==
  data: acc_vec input; euler_angles output; Psi input; acc_res output
function [euler_angles, acc_res] = fcn(acc_vec, Psi) %#codegen
[euler_angles, acc_res] = ...
    getEulerAnglesFromAccelerationVectorAndHeading(acc_vec, Psi);
end

== matlab function multicopterNDI_lib/Horizontal INDI position (NE) controller cascade with reduced attitude increment (quaternion) command/MATLAB Function2 ==
  data: q_cmd_red output; phi input; delta input
function q_cmd_red  = fcn(phi,delta)

x = sin(delta);
y = -cos(delta);

xy = sqrt(x^2+y^2);
if xy <= 1e-2
    x = single(1);
    xy_save = sqrt(x^2+y^2);
else
    xy_save = xy;
end
n_d_red = 1/xy_save*[x;y;0];

% [1] eq. (1)
q_0 = cos(phi/2);
q_t = n_d_red * sin(phi/2);
q_cmd_red = [q_0;q_t];

end

== matlab function multicopterNDI_lib/Horizontal INDI position (FR) controller cascade/MATLAB Function ==
  data: xy_b_ddt_cmd input; B_inv output; acc_vertical_measure input; Theta input
function B_inv = fcn(xy_b_ddt_cmd,acc_vertical_measure,Theta) %#codegen
    [Phi_dAcc,Theta_dAcc] = eulerAngles_dAcc(xy_b_ddt_cmd,acc_vertical_measure,Theta);
    B_inv = [ Phi_dAcc; Theta_dAcc ];
end

== matlab function multicopterNDI_lib/Horizontal INDI position (FR) controller cascade/filtered command/MATLAB Function ==
  data: V_FR input; V_NE output; Psi input
function V_NE = fcn(V_FR,Psi)

V_NE = [ cos(Psi), -sin(Psi); sin(Psi), cos(Psi) ] * V_FR;

end

== matlab function multicopterNDI_lib/Horizontal INDI position (NE) controller cascade with reduced attitude increment (quaternion) command/MATLAB Function8 ==
  data: q_cmd_red output; phi input; delta input
function q_cmd_red  = fcn(phi,delta)

x = sin(delta);
y = -cos(delta);

xy = sqrt(x^2+y^2);
if xy <= 1e-2
    x = single(1);
    xy_save = sqrt(x^2+y^2);
else
    xy_save = xy;
end
n_d_red = 1/xy_save*[x;y;0];

% [1] eq. (1)
q_0 = cos(phi/2);
q_t = n_d_red * sin(phi/2);
q_cmd_red = [q_0;q_t];

end

== matlab function multicopterNDI_lib/Horizontal NDI position (NE) controller cascade with reduced attitude (angle) command/MATLAB Function1 ==
  data: phi output; delta output; xyz_g_dt2 input
function [phi,delta] = fcn(xyz_g_dt2)

if abs(xyz_g_dt2(3)) < 1
    if xyz_g_dt2(3) > 0
        xyz_g_dt2(3) = 1;
    else
        xyz_g_dt2(3) = -1;
    end
end


delta = atan2(xyz_g_dt2(2),xyz_g_dt2(1));
xy_g_dt2 = sqrt( xyz_g_dt2(1)^2 + xyz_g_dt2(2)^2 );
phi = atan2( xy_g_dt2 , -xyz_g_dt2(3) );

end

== matlab function multicopterNDI_lib/Horizontal INDI position (NE) controller cascade with reduced attitude increment (quaternion) command/MATLAB Function9 ==
  data: phi output; delta output; xyz_g_dt2 input
function [phi,delta] = fcn(xyz_g_dt2)
% function [x,y] = fcn(xyz_g_dt2)

if abs(xyz_g_dt2(3)) < 1
    if xyz_g_dt2(3) > 0
        xyz_g_dt2(3) = 1;
    else
        xyz_g_dt2(3) = -1;
    end
end

% x = atan2(xyz_g_dt2(1),-xyz_g_dt2(3));
% y = atan2(xyz_g_dt2(2),-xyz_g_dt2(3));


delta = atan2(xyz_g_dt2(2),xyz_g_dt2(1));
xy_g_dt2 = sqrt( xyz_g_dt2(1)^2 + xyz_g_dt2(2)^2 );
phi = atan2( xy_g_dt2 , -xyz_g_dt2(3) );

end

== matlab function multicopterNDI_lib/Horizontal INDI position (NE) controller cascade with reduced attitude increment (quaternion) command/MATLAB Function11 ==
  data: q_cmd input; q_e output; q_m input
function q_e = fcn(q_cmd, q_m)

q_e = quatMultiply(quatInv(q_m),q_cmd);
